simulink model "SistemaPF"  (R2023a)
settings: Solver=VariableStepAuto  StartTime=0.0  StopTime=10.0  MaxStep=1e-3  RelTol=1e-3
libraries: fl_lib x20, nesl_utility x6, slpidlib x1
settings Model: Creator=gabri  LastModifiedBy=gabri
settings DataIOCC: SaveOutput=off  SignalLogging=off  DSMLogging=off  ReturnWorkspaceOutputs=off  TimeSaveName=t
settings DebuggingCC: AlgebraicLoopMsg=none  ArtificialAlgebraicLoopMsg=none  MaxConsecutiveZCsMsg=none  ModelReferenceExtraNoncontSigs=none  OperatingPointInterfaceChecksumMismatchMsg=none

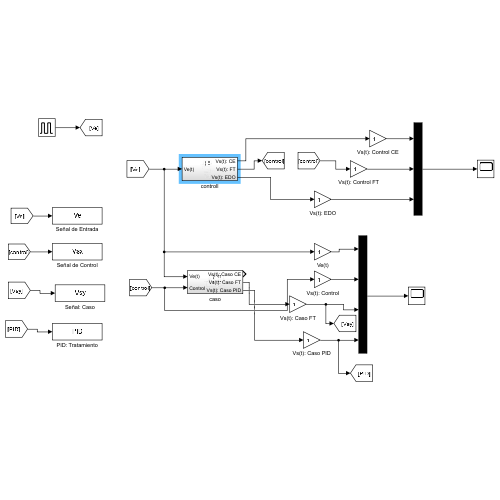
[thumbnail: Simulink's stored preview of the top-level diagram]
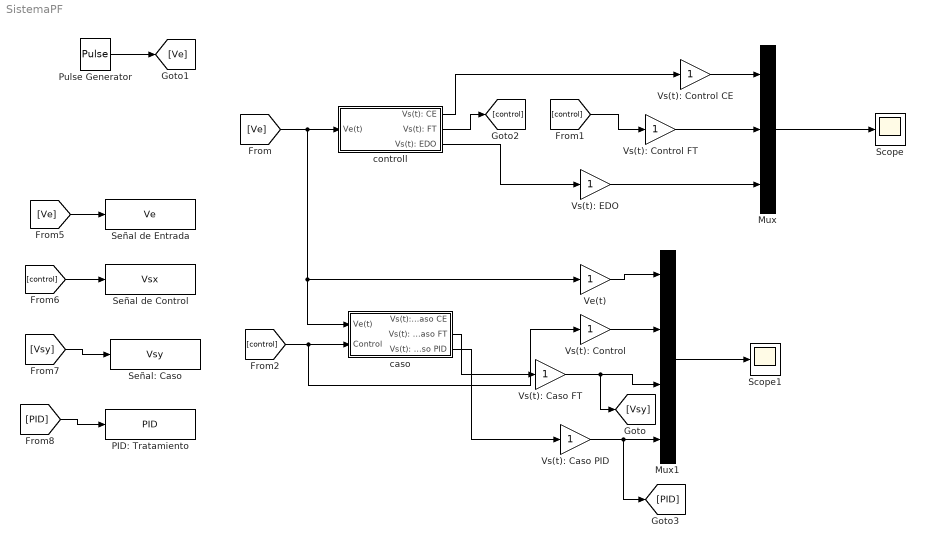
== system SistemaPF ==
  Mux : Mux  Inputs=3
  Mux1 : Mux
  PID: Tratamiento : ToWorkspace  VariableName=PID  SampleTime=-1
  Pulse Generator : DiscretePulseGenerator  PulseType=Time based  Period=15  PulseWidth=20  PhaseDelay=1
  Scope : Scope
  Scope1 : Scope
  Señal de Control : ToWorkspace  VariableName=Vsx  SampleTime=-1
  Señal de Entrada : ToWorkspace  VariableName=Ve  SampleTime=-1
  Señal: Caso : ToWorkspace  VariableName=Vsy  SampleTime=-1
  Ve(t) : Gain
  Vs(t): Caso FT : Gain
  Vs(t): Caso PID : Gain
  Vs(t): Control : Gain
  Vs(t): Control CE : Gain
  Vs(t): Control FT : Gain
  Vs(t): EDO : Gain
  caso : Subsystem
  controll : Subsystem
  wires:
  Mux/1 -> Scope/1
  Pulse Generator/1 -> [Ve]
  [Ve] -> caso/1(Ve(t)), Ve(t)/1, controll/1(Ve(t))
  controll/2(Vs(t): FT) -> [control]
  Vs(t): Control FT/1 -> Mux/2
  [control] -> Vs(t): Control FT/1
  controll/3(Vs(t): EDO) -> Vs(t): EDO/1
  Vs(t): EDO/1 -> Mux/3
  Mux1/1 -> Scope1/1
  [control] -> Vs(t): Control/1, caso/2(Control)
  caso/2(Vs(t): Caso FT) -> Vs(t): Caso FT/1
  Vs(t): Control CE/1 -> Mux/1
  controll/1(Vs(t): CE) -> Vs(t): Control CE/1
  Ve(t)/1 -> Mux1/1
  Vs(t): Caso FT/1 -> [Vsy], Mux1/3
  Vs(t): Control/1 -> Mux1/2
  Vs(t): Caso PID/1 -> [PID], Mux1/4
  caso/3(Vs(t): Caso PID) -> Vs(t): Caso PID/1
  [PID] -> PID: Tratamiento/1
  [Vsy] -> Señal: Caso/1
  [control] -> Señal de Control/1
  [Ve] -> Señal de Entrada/1

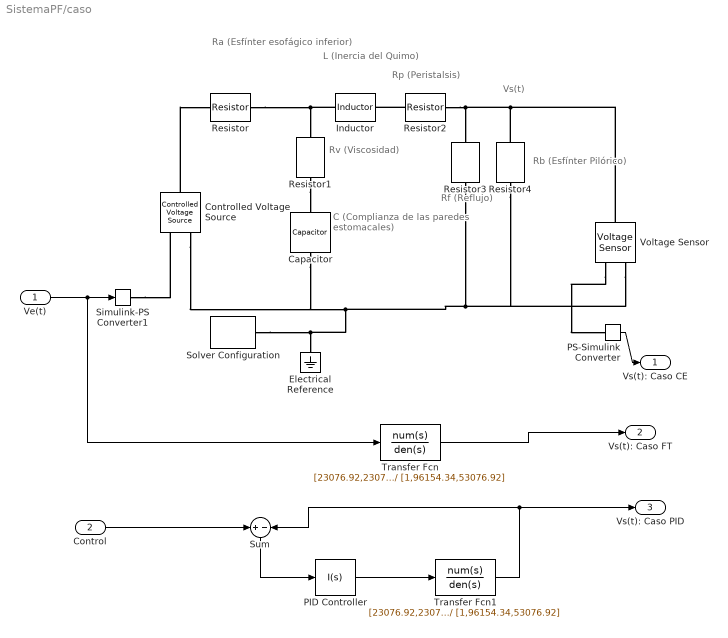
== system SistemaPF/caso ==
  note: C (Complianza de las paredes estomacales)
  note: Rv
      | (Viscosidad)
  note: Rf (Reflujo)
  note: Rb (Esfínter Pilórico)
  note: Rp (Peristalsis)
  note: L (Inercia del Quimo)
  note: Vs(t)
  note: Ra
      | (Esfínter esofágico inferior)
  Ve(t) : Inport
  Control : Inport  Port=2
  Capacitor : fl_lib/Electrical/Electrical Elements/Capacitor  c=100e-6 F  r=1e-6 Ohm  g=0 1/Ohm  i_specify=off  i_priority=None  i=0 A  i_nominal_specify=off  i_nominal_unit=A  i_nominal_value=1  v_specify=off  v_priority=None  v=0 V  v_nominal_specify=off  v_nominal_unit=V  v_nominal_value=1  vc_specify=off  vc_priority=High  vc=0 V  vc_nominal_specify=off  vc_nominal_unit=V  vc_nominal_value=1
  Controlled Voltage Source : fl_lib/Electrical/Electrical Sources/Controlled Voltage Source
  Electrical Reference : fl_lib/Electrical/Electrical Elements/Electrical Reference
  Inductor : fl_lib/Electrical/Electrical Elements/Inductor  l=500e-3 H  r=0 Ohm  g=1e-9 1/Ohm  i_specify=off  i_priority=None  i=0 A  i_nominal_specify=off  i_nominal_unit=A  i_nominal_value=1  v_specify=off  v_priority=None  v=0 V  v_nominal_specify=off  v_nominal_unit=V  v_nominal_value=1  i_L_specify=off  i_L_priority=High  i_L=0 A  i_L_nominal_specify=off  i_L_nominal_unit=A  i_L_nominal_value=1
  PID Controller : slpidlib/PID Controller  Controller=I  Form=Parallel  TimeDomain=Continuous-time  UseExternalTs=off  SampleTime=-1  IntegratorMethod=Forward Euler  FilterMethod=Forward Euler  ControllerParametersSource=internal  P=0  I=1666.67668082261  UseKiTs=off  D=0  N=100  UseFilter=on  TunerSelectOption=Transfer Function Based (PID Tuner App)  InitialConditionSource=internal  InitialConditionForIntegrator=0  InitialConditionForFilter=0  DifferentiatorICPrevScaledInput=0  ExternalReset=none  TrackingMode=off  Kt=1  LimitOutput=off  SatLimitsSource=internal  UpperSaturationLimit=inf  LowerSaturationLimit=-inf  LinearizeAsGain=on  AntiWindupMode=none  Kb=1  LimitIntegrator=off  UpperIntegratorSaturationLimit=inf  LowerIntegratorSaturationLimit=-inf  POutMin=[]  POutMax=[]  IOutMin=[]  IOutMax=[]  DOutMin=[]  DOutMax=[]  NOutMin=[]  NOutMax=[]  SumOutMin=[]  SumOutMax=[]  SaturationOutMin=[]  SaturationOutMax=[]  PParamMin=[]  PParamMax=[]  IParamMin=[]  IParamMax=[]  DParamMin=[]  DParamMax=[]  NParamMin=[]  NParamMax=[]  KbParamMin=[]  KbParamMax=[]  KtParamMin=[]  KtParamMax=[]  KbOutMin=[]  KbOutMax=[]  KtOutMin=[]  KtOutMax=[]  IntegratorOutMin=[]  IntegratorOutMax=[]  FilterOutMin=[]  FilterOutMax=[]  SumI1OutMin=[]  SumI1OutMax=[]  SumI2OutMin=[]  SumI2OutMax=[]  SumI3OutMin=[]  SumI3OutMax=[]  SumI4OutMin=[]  SumI4OutMax=[]  SumDOutMin=[]  SumDOutMax=[]  DifferentiatorOutMin=[]  DifferentiatorOutMax=[]  FilterDiffOutCoefMin=[]  FilterDiffOutCoefMax=[]  ReciprocalOutMin=[]  ReciprocalOutMax=[]  SumDenOutMin=[]  SumDenOutMax=[]  SumNumOutMin=[]  SumNumOutMax=[]  DivideOutMin=[]  DivideOutMax=[]  UdiffTsProdOutMin=[]  UdiffTsProdOutMax=[]  NTsProdOutMin=[]  NTsProdOutMax=[]  UintegralTsProdOutMin=[]  UintegralTsProdOutMax=[]  UngainTsProdOutMin=[]  UngainTsProdOutMax=[]  ClampingZeroOutDataTypeStr=Inherit: Inherit via back propagation  ClampingZeroOutMin=[]  ClampingZeroOutMax=[]  FilterDenConstantOutDataTypeStr=Inherit: Inherit via back propagation  FilterDenConstantOutMin=[]  FilterDenConstantOutMax=[]  PCopyOutDataTypeStr=Inherit: Inherit via back propagation  PCopyOutMin=[]  PCopyOutMax=[]  NCopyOutDataTypeStr=Inherit: Inherit via back propagation  NCopyOutMin=[]  NCopyOutMax=[]  IntegratorContinuousStateAttributes=''  IntegratorStateMustResolveToSignalObject=off  IntegratorRTWStateStorageClass=Auto  FilterContinuousStateAttributes=''  FilterStateMustResolveToSignalObject=off  FilterRTWStateStorageClass=Auto  ParallelPVariant=Disabled  IdealPVariant=Disabled  IVariant=InternalParameters  DVariant=Disabled  IntegratorVariant=Continuous  SatVariant=Disabled  AWVariant=Passthrough  PCopyVariant=Disabled  TRVariant=Disabled  FdbkBlocksVariant=Forward  IdealPFdbkVariant=Disabled  SatFdbkVariant=Disabled  DerivativeFilterVariant=Disabled  NVariant=Disabled  NCopyVariant=Disabled_SignalSpec  FilterICVariant=Disabled  IntegratorICVariant=InternalICs  ExternalResetVariant=Disabled  TRSumVariant=Passthrough  SumFdbkVariant=Disabled  SumVariant=Passthrough_I  TsampFilterVariant=InternalTs  TsampNgainVariant=Passthrough  TsampIntegralVariant=Disabled_SignalSpec  ExternalSaturationOutDataTypeStr=Inherit: Same as second input
  PS-Simulink Converter : nesl_utility/PS-Simulink Converter  PhysicalDomain=network_engine_domain  SubClassName=ps_output  LeftPortType=input  RightPortType=output  PseudoPeriodic=off  Frequencies=[]  VectorFormat=inherit  Unit=inherit  AffineConversion=off
  Resistor : fl_lib/Electrical/Electrical Elements/Resistor  R=10 kOhm  i_specify=off  i_priority=None  i=0 A  i_nominal_specify=off  i_nominal_unit=A  i_nominal_value=1  v_specify=off  v_priority=None  v=0 V  v_nominal_specify=off  v_nominal_unit=V  v_nominal_value=1
  Resistor1 : fl_lib/Electrical/Electrical Elements/Resistor  R=10 kOhm  i_specify=off  i_priority=None  i=0 A  i_nominal_specify=off  i_nominal_unit=A  i_nominal_value=1  v_specify=off  v_priority=None  v=0 V  v_nominal_specify=off  v_nominal_unit=V  v_nominal_value=1
  Resistor2 : fl_lib/Electrical/Electrical Elements/Resistor  R=20 kOhm  i_specify=off  i_priority=None  i=0 A  i_nominal_specify=off  i_nominal_unit=A  i_nominal_value=1  v_specify=off  v_priority=None  v=0 V  v_nominal_specify=off  v_nominal_unit=V  v_nominal_value=1
  Resistor3 : fl_lib/Electrical/Electrical Elements/Resistor  R=30 kOhm  i_specify=off  i_priority=None  i=0 A  i_nominal_specify=off  i_nominal_unit=A  i_nominal_value=1  v_specify=off  v_priority=None  v=0 V  v_nominal_specify=off  v_nominal_unit=V  v_nominal_value=1
  Resistor4 : fl_lib/Electrical/Electrical Elements/Resistor  R=100 kOhm  i_specify=off  i_priority=None  i=0 A  i_nominal_specify=off  i_nominal_unit=A  i_nominal_value=1  v_specify=off  v_priority=None  v=0 V  v_nominal_specify=off  v_nominal_unit=V  v_nominal_value=1
  Simulink-PS Converter1 : nesl_utility/Simulink-PS Converter  PhysicalDomain=network_engine_domain  SubClassName=ps_input  LeftPortType=input  RightPortType=output  PseudoPeriodic=off  Frequencies=[]  NoiseDistribution=none  NoiseParameters=[]  Unit=1  AffineConversion=off  FilteringAndDerivatives=provide  SimscapeFilterOrder=1  InputFilterTimeConstant=0.001  UdotUserProvided=0
  Solver Configuration : nesl_utility/Solver Configuration  PhysicalDomain=network_engine_domain  SubClassName=solver  LeftPortType=input  RightPortType=generic  Tones=[]  Harmonics=[]  SimulateNoise=off  Profile=off  UseLocalSampling=off  EnableSwitchedLinearOptims=on  FrequencyDomain=off  UseCCode=off  RelTol=0.001  AbsTol=0.001  MinStep=1e-09  ToWorkspace=off  RevertToSquareIcSolve=off  NumHomotopyIterations=100  PhasorMode=off  PhasorModeNumHarmonics=1  ConsistencySolver=NEWTON_XTOL_AFTER_FTOL  IndexReductionMethod=DerivativeReplacement  DoDC=off  ResidualTolerance=1e-09  ConsistencyTolSource=GLOBAL  ConsistencyAbsTol=0.001  ConsistencyRelTol=0.001  ConsistencyTolFactor=0.001  UseLocalSolver=off  LocalSolverChoice=NE_BACKWARD_EULER_ADVANCER  ResolveIndetEquations=on  FunctionEvalNumThread=1  LocalSolverSampleTime=0.001  DoFixedCost=off  MaxNonlinIter=3  MaxModeIter=2  ComputeImpulses=off  ImpulseIterations=2  LinearAlgebra=auto  LinearAlgebraNumThread=0  EquationFormulation=NE_TIME_EF  DelaysMemoryBudget=1024  AutomaticFiltering=on  FilteringTimeConstant=0.001  PartitionStorageMethod=AS_NEEDED  PartitionMemoryBudget=1024  PartitionMethod=ROBUST
  Sum : Sum  Inputs=+-
  Transfer Fcn : TransferFcn  Numerator=[23076.92,23076.92]  Denominator=[1,96154.34,53076.92]
  Transfer Fcn1 : TransferFcn  Numerator=[23076.92,23076.92]  Denominator=[1,96154.34,53076.92]
  Voltage Sensor : fl_lib/Electrical/Electrical Sensors/Voltage Sensor
  Vs(t): Caso CE : Outport
  Vs(t): Caso FT : Outport  Port=2
  Vs(t): Caso PID : Outport  Port=3
  wires:
  Ve(t)/1 -> Transfer Fcn/1, Simulink-PS Converter1/1
  PS-Simulink Converter/1 -> Vs(t): Caso CE/1
  Transfer Fcn/1 -> Vs(t): Caso FT/1
  Sum/1 -> PID Controller/1
  PID Controller/1 -> Transfer Fcn1/1
  Transfer Fcn1/1 -> Vs(t): Caso PID/1, Sum/2
  Control/1 -> Sum/1
  connections:
  Resistor4/LConn1 -- Voltage Sensor/LConn1 -- Resistor2/RConn1 -- Resistor3/LConn1
  Resistor/RConn1 -- Inductor/LConn1 -- Resistor1/LConn1
  Resistor3/RConn1 -- Resistor4/RConn1 -- Voltage Sensor/RConn2 -- Capacitor/RConn1 -- Controlled Voltage Source/RConn2 -- Solver Configuration/RConn1 -- Electrical Reference/LConn1
  Resistor1/RConn1 -- Capacitor/LConn1
  Simulink-PS Converter1/RConn1 -- Controlled Voltage Source/RConn1
  Voltage Sensor/RConn1 -- PS-Simulink Converter/LConn1
  Controlled Voltage Source/LConn1 -- Resistor/LConn1
  Resistor2/LConn1 -- Inductor/RConn1

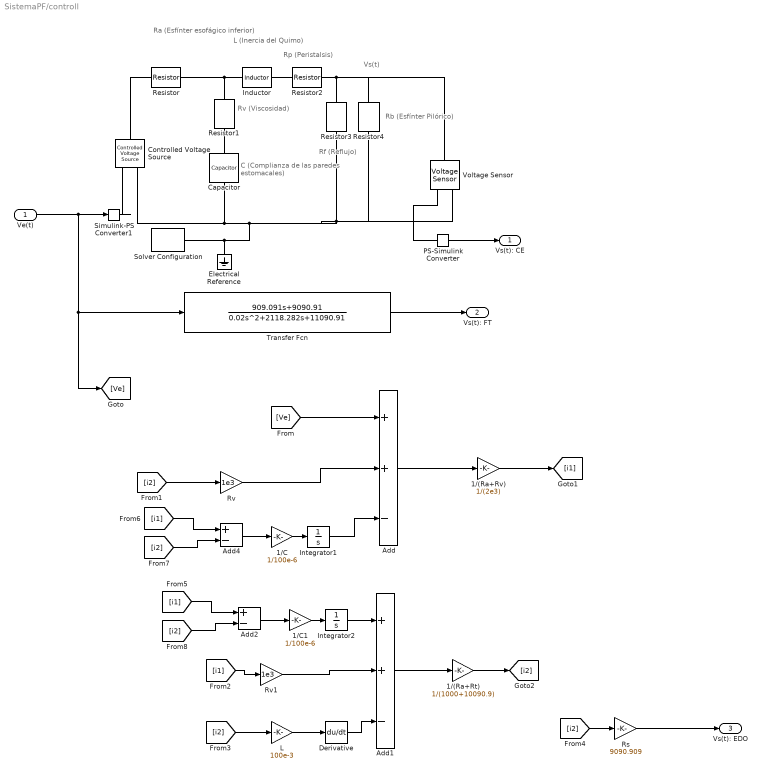
== system SistemaPF/controll ==
  note: Rb (Esfínter Pilórico)
  note: Rf (Reflujo)
  note: Rp (Peristalsis)
  note: C (Complianza de las paredes estomacales)
  note: Rv
      | (Viscosidad)
  note: Vs(t)
  note: L (Inercia del Quimo)
  note: Ra
      | (Esfínter esofágico inferior)
  Ve(t) : Inport
  1/(Ra+Rt) : Gain  Gain=1/(1000+10090.9)
  1/(Ra+Rv) : Gain  Gain=1/(2e3)
  1/C : Gain  Gain=1/100e-6
  1/C1 : Gain  Gain=1/100e-6
  Add : Sum  Inputs=++-
  Add1 : Sum  Inputs=++-
  Add2 : Sum  Inputs=+-
  Add4 : Sum  Inputs=+-
  Capacitor : fl_lib/Electrical/Electrical Elements/Capacitor  c=100e-6 F  r=1e-6 Ohm  g=0 1/Ohm  i_specify=off  i_priority=None  i=0 A  i_nominal_specify=off  i_nominal_unit=A  i_nominal_value=1  v_specify=off  v_priority=None  v=0 V  v_nominal_specify=off  v_nominal_unit=V  v_nominal_value=1  vc_specify=off  vc_priority=High  vc=0 V  vc_nominal_specify=off  vc_nominal_unit=V  vc_nominal_value=1
  Controlled Voltage Source : fl_lib/Electrical/Electrical Sources/Controlled Voltage Source
  Derivative : Derivative
  Electrical Reference : fl_lib/Electrical/Electrical Elements/Electrical Reference
  Inductor : fl_lib/Electrical/Electrical Elements/Inductor  l=100e-3 H  r=0 Ohm  g=1e-9 1/Ohm  i_specify=off  i_priority=None  i=0 A  i_nominal_specify=off  i_nominal_unit=A  i_nominal_value=1  v_specify=off  v_priority=None  v=0 V  v_nominal_specify=off  v_nominal_unit=V  v_nominal_value=1  i_L_specify=off  i_L_priority=High  i_L=0 A  i_L_nominal_specify=off  i_L_nominal_unit=A  i_L_nominal_value=1
  Integrator1 : Integrator
  Integrator2 : Integrator
  L : Gain  Gain=100e-3
  PS-Simulink Converter : nesl_utility/PS-Simulink Converter  PhysicalDomain=network_engine_domain  SubClassName=ps_output  LeftPortType=input  RightPortType=output  PseudoPeriodic=off  Frequencies=[]  VectorFormat=inherit  Unit=inherit  AffineConversion=off
  Resistor : fl_lib/Electrical/Electrical Elements/Resistor  R=1 kOhm  i_specify=off  i_priority=None  i=0 A  i_nominal_specify=off  i_nominal_unit=A  i_nominal_value=1  v_specify=off  v_priority=None  v=0 V  v_nominal_specify=off  v_nominal_unit=V  v_nominal_value=1
  Resistor1 : fl_lib/Electrical/Electrical Elements/Resistor  R=1 kOhm  i_specify=off  i_priority=None  i=0 A  i_nominal_specify=off  i_nominal_unit=A  i_nominal_value=1  v_specify=off  v_priority=None  v=0 V  v_nominal_specify=off  v_nominal_unit=V  v_nominal_value=1
  Resistor2 : fl_lib/Electrical/Electrical Elements/Resistor  R=1 kOhm  i_specify=off  i_priority=None  i=0 A  i_nominal_specify=off  i_nominal_unit=A  i_nominal_value=1  v_specify=off  v_priority=None  v=0 V  v_nominal_specify=off  v_nominal_unit=V  v_nominal_value=1
  Resistor3 : fl_lib/Electrical/Electrical Elements/Resistor  R=100 kOhm  i_specify=off  i_priority=None  i=0 A  i_nominal_specify=off  i_nominal_unit=A  i_nominal_value=1  v_specify=off  v_priority=None  v=0 V  v_nominal_specify=off  v_nominal_unit=V  v_nominal_value=1
  Resistor4 : fl_lib/Electrical/Electrical Elements/Resistor  R=10 kOhm  i_specify=off  i_priority=None  i=0 A  i_nominal_specify=off  i_nominal_unit=A  i_nominal_value=1  v_specify=off  v_priority=None  v=0 V  v_nominal_specify=off  v_nominal_unit=V  v_nominal_value=1
  Rs : Gain  Gain=9090.909
  Rv : Gain  Gain=1e3
  Rv1 : Gain  Gain=1e3
  Simulink-PS Converter1 : nesl_utility/Simulink-PS Converter  PhysicalDomain=network_engine_domain  SubClassName=ps_input  LeftPortType=input  RightPortType=output  PseudoPeriodic=off  Frequencies=[]  NoiseDistribution=none  NoiseParameters=[]  Unit=1  AffineConversion=off  FilteringAndDerivatives=provide  SimscapeFilterOrder=1  InputFilterTimeConstant=0.001  UdotUserProvided=0
  Solver Configuration : nesl_utility/Solver Configuration  PhysicalDomain=network_engine_domain  SubClassName=solver  LeftPortType=input  RightPortType=generic  Tones=[]  Harmonics=[]  SimulateNoise=off  Profile=off  UseLocalSampling=off  EnableSwitchedLinearOptims=on  FrequencyDomain=off  UseCCode=off  RelTol=0.001  AbsTol=0.001  MinStep=1e-09  ToWorkspace=off  RevertToSquareIcSolve=off  NumHomotopyIterations=100  PhasorMode=off  PhasorModeNumHarmonics=1  ConsistencySolver=NEWTON_XTOL_AFTER_FTOL  IndexReductionMethod=DerivativeReplacement  DoDC=off  ResidualTolerance=1e-09  ConsistencyTolSource=GLOBAL  ConsistencyAbsTol=0.001  ConsistencyRelTol=0.001  ConsistencyTolFactor=0.001  UseLocalSolver=off  LocalSolverChoice=NE_BACKWARD_EULER_ADVANCER  ResolveIndetEquations=on  FunctionEvalNumThread=1  LocalSolverSampleTime=0.001  DoFixedCost=off  MaxNonlinIter=3  MaxModeIter=2  ComputeImpulses=off  ImpulseIterations=2  LinearAlgebra=auto  LinearAlgebraNumThread=0  EquationFormulation=NE_TIME_EF  DelaysMemoryBudget=1024  AutomaticFiltering=on  FilteringTimeConstant=0.001  PartitionStorageMethod=AS_NEEDED  PartitionMemoryBudget=1024  PartitionMethod=ROBUST
  Transfer Fcn : TransferFcn  Numerator=[909.091,9090.91]  Denominator=[0.02,2118.282,11090.91]
  Voltage Sensor : fl_lib/Electrical/Electrical Sensors/Voltage Sensor
  Vs(t): CE : Outport
  Vs(t): FT : Outport  Port=2
  Vs(t): EDO : Outport  Port=3
  wires:
  Ve(t)/1 -> [Ve], Transfer Fcn/1, Simulink-PS Converter1/1
  PS-Simulink Converter/1 -> Vs(t): CE/1
  Transfer Fcn/1 -> Vs(t): FT/1
  [Ve] -> Add/1
  [i2] -> Rv/1
  Rv/1 -> Add/2
  [i2] -> Add4/2
  Add4/1 -> 1/C/1
  1/C/1 -> Integrator1/1
  [i1] -> Add4/1
  Integrator1/1 -> Add/3
  Add/1 -> 1/(Ra+Rv)/1
  1/(Ra+Rv)/1 -> [i1]
  [i1] -> Rv1/1
  Rv1/1 -> Add1/2
  L/1 -> Derivative/1
  [i2] -> L/1
  Derivative/1 -> Add1/3
  Add1/1 -> 1/(Ra+Rt)/1
  1/(Ra+Rt)/1 -> [i2]
  [i2] -> Rs/1
  Rs/1 -> Vs(t): EDO/1
  [i1] -> Add2/1
  1/C1/1 -> Integrator2/1
  Add2/1 -> 1/C1/1
  [i2] -> Add2/2
  Integrator2/1 -> Add1/1
  connections:
  Controlled Voltage Source/LConn1 -- Resistor/LConn1
  Simulink-PS Converter1/RConn1 -- Controlled Voltage Source/RConn1
  Voltage Sensor/RConn1 -- PS-Simulink Converter/LConn1
  Resistor2/RConn1 -- Voltage Sensor/LConn1 -- Resistor4/LConn1 -- Resistor3/LConn1
  Capacitor/RConn1 -- Resistor4/RConn1 -- Voltage Sensor/RConn2 -- Resistor3/RConn1 -- Solver Configuration/RConn1 -- Electrical Reference/LConn1 -- Controlled Voltage Source/RConn2
  Resistor1/RConn1 -- Capacitor/LConn1
  Resistor/RConn1 -- Inductor/LConn1 -- Resistor1/LConn1
  Resistor2/LConn1 -- Inductor/RConn1
